simulink model "OpenXstim_B2B4_PI"  (R2025a)
settings: Solver=FixedStepDiscrete  StartTime=0  StopTime=62.106999999999999  FixedStep=0.08249999999999999  RelTol=1e-3
settings Model: Creator=arnav  LastModifiedBy=arnav

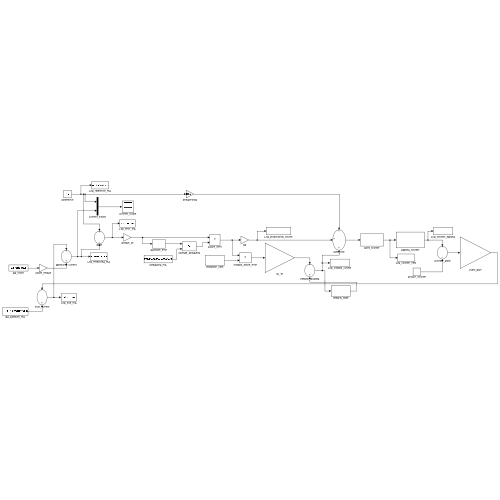
[thumbnail: Simulink's stored preview of the top-level diagram]
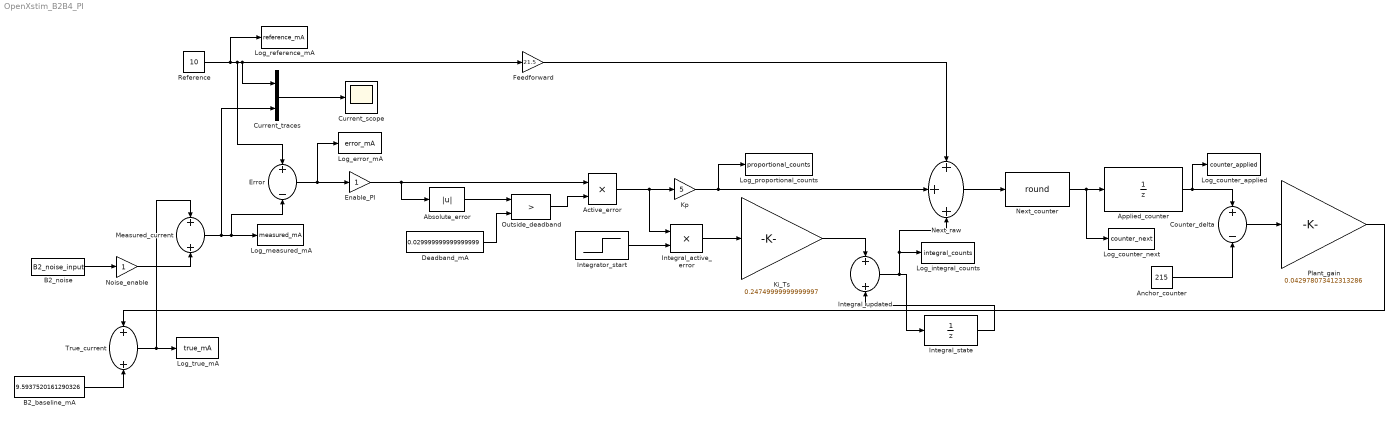
== system OpenXstim_B2B4_PI ==
  Absolute_error : Abs  SaturateOnIntegerOverflow=off
  Active_error : Product
  Anchor_counter : Constant  Value=215
  Applied_counter : UnitDelay  InitialCondition=215  SampleTime=0.08249999999999999  HasFrameUpgradeWarning=on
  B2_baseline_mA : Constant  Value=9.5937520161290326
  B2_noise : FromWorkspace  VariableName=B2_noise_input  Interpolate=off  OutputAfterFinalValue=Holding final value
  Counter_delta : Sum  Inputs=+-
  Current_scope : Scope
  Current_traces : Mux  Inputs=2
  Deadband_mA : Constant  Value=0.029999999999999999
  Enable_PI : Gain
  Error : Sum  Inputs=+-
  Feedforward : Gain  Gain=21.5
  Integral_active_error : Product
  Integral_state : UnitDelay  SampleTime=0.08249999999999999  HasFrameUpgradeWarning=on
  Integral_updated : Sum
  Integrator_start : Step  Time=0.041249999999999995  SampleTime=0
  Ki_Ts : Gain  Gain=0.24749999999999997
  Kp : Gain  Gain=5
  Log_counter_applied : ToWorkspace  VariableName=counter_applied  SaveFormat=Timeseries  SampleTime=-1
  Log_counter_next : ToWorkspace  VariableName=counter_next  SaveFormat=Timeseries  SampleTime=-1
  Log_error_mA : ToWorkspace  VariableName=error_mA  SaveFormat=Timeseries  SampleTime=-1
  Log_integral_counts : ToWorkspace  VariableName=integral_counts  SaveFormat=Timeseries  SampleTime=-1
  Log_measured_mA : ToWorkspace  VariableName=measured_mA  SaveFormat=Timeseries  SampleTime=-1
  Log_proportional_counts : ToWorkspace  VariableName=proportional_counts  SaveFormat=Timeseries  SampleTime=-1
  Log_reference_mA : ToWorkspace  VariableName=reference_mA  SaveFormat=Timeseries  SampleTime=-1
  Log_true_mA : ToWorkspace  VariableName=true_mA  SaveFormat=Timeseries  SampleTime=-1
  Measured_current : Sum
  Next_counter : Rounding  Operator=round
  Next_raw : Sum  Inputs=+++
  Noise_enable : Gain
  Outside_deadband : RelationalOperator  Operator=>  OutDataTypeStr=boolean  RndMeth=Simplest  InputSameDT=off
  Plant_gain : Gain  Gain=0.042978073412313286
  Reference : Constant  Value=10
  True_current : Sum
  wires:
  Plant_gain/1 -> True_current/1
  Counter_delta/1 -> Plant_gain/1
  Anchor_counter/1 -> Counter_delta/2
  B2_noise/1 -> Noise_enable/1
  Integral_state/1 -> Integral_updated/2
  Enable_PI/1 -> Absolute_error/1, Active_error/1
  Next_raw/1 -> Next_counter/1
  Integrator_start/1 -> Integral_active_error/2
  Applied_counter/1 -> Log_counter_applied/1, Counter_delta/1
  Active_error/1 -> Integral_active_error/1, Kp/1
  Outside_deadband/1 -> Active_error/2
  Feedforward/1 -> Next_raw/1
  Ki_Ts/1 -> Integral_updated/1
  Error/1 -> Log_error_mA/1, Enable_PI/1
  Integral_updated/1 -> Log_integral_counts/1, Next_raw/3, Integral_state/1
  Noise_enable/1 -> Measured_current/2
  Current_traces/1 -> Current_scope/1
  Kp/1 -> Log_proportional_counts/1, Next_raw/2
  Measured_current/1 -> Log_measured_mA/1, Error/2, Current_traces/2
  Integral_active_error/1 -> Ki_Ts/1
  B2_baseline_mA/1 -> True_current/2
  True_current/1 -> Log_true_mA/1, Measured_current/1
  Next_counter/1 -> Log_counter_next/1, Applied_counter/1
  Absolute_error/1 -> Outside_deadband/1
  Reference/1 -> Current_traces/1, Feedforward/1, Error/1, Log_reference_mA/1
  Deadband_mA/1 -> Outside_deadband/2
